simulink model "rp_spectrometer_v2"  (R2022a)
settings: Solver=FixedStepDiscrete  StartTime=0.0  StopTime=4194304  RelTol=1e-3
undefined symbols (not defined in the file): xc7z010clg400
libraries: hdlBasic x93, casper_library_misc x4, vmcUtilities x1, xps_library x1
(part 2 of 2)

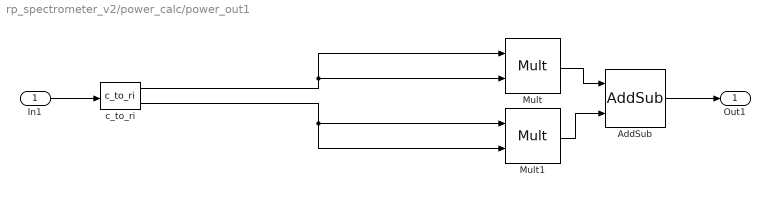
== system rp_spectrometer_v2/power_calc/power_out1 ==
  In1 : Inport
  AddSub : hdlBasic/AddSub  mode=Addition  use_carryin=off  use_carryout=off  en=off  latency=0  precision=Full  arith_type=Unsigned  n_bits=16  bin_pt=14  quantization=Truncate  overflow=Wrap  use_behavioral_HDL=off  hw_selection=Fabric  pipelined=off  XmcBlockStatus=1  maskContainerNames=tabcontainer1  block_type=addsub  block_config=sysgen:Addsub_config
  Mult : hdlBasic/Mult  precision=User Defined  arith_type="Signed  (2's comp)"  n_bits=32  bin_pt=30  quantization=Truncate  overflow=Wrap  en=off  latency=0  use_behavioral_HDL=off  opt=Speed  use_embedded=on  optimum_pipeline=off  pipeline=on  use_rpm=on  placement_style=Triangular  XmcBlockStatus=1  maskContainerNames=group1  block_type=mult  block_config=sysgen:Mult_config  block_width=598  block_height=876
  Mult1 : hdlBasic/Mult  precision=User Defined  arith_type="Signed  (2's comp)"  n_bits=32  bin_pt=30  quantization=Truncate  overflow=Wrap  en=off  latency=0  use_behavioral_HDL=off  opt=Speed  use_embedded=on  optimum_pipeline=off  pipeline=on  use_rpm=on  placement_style=Triangular  XmcBlockStatus=1  maskContainerNames=group1  block_type=mult  block_config=sysgen:Mult_config  block_width=598  block_height=876
  c_to_ri : casper_library_misc/c_to_ri  n_bits=14  bin_pt=13
      settings: AttributesFormatString=14_13 r/i  SourceProductName=CASPER DSP Blockset
  Out1 : Outport  VectorParamsAs1DForOutWhenUnconnected=off
  wires:
  Mult1/1 -> AddSub/2
  Mult/1 -> AddSub/1
  AddSub/1 -> Out1/1
  In1/1 -> c_to_ri/1
  c_to_ri/1 -> Mult/2, Mult/1
  c_to_ri/2 -> Mult1/1, Mult1/2

== system rp_spectrometer_v2/simple_bram_vacc/delay_bram ==
  In1 : Inport
  Constant2 : hdlBasic/Constant  const=1  gui_display_data_type=Boolean  arith_type=Boolean  n_bits=1  bin_pt=0  preci_type=Single  exp_width=8  frac_width=24  explicit_period=on  period=1  XmcBlockStatus=1  maskContainerNames=tabcontainer1  block_type=constant  block_config=sysgen:Constant_config
  Counter : hdlBasic/Counter  cnt_type=Count limited  cnt_to=DelayLen - bram_latency - 1  operation=Up  start_count=0  cnt_by_val=1  arith_type=Unsigned  n_bits=BitWidth  bin_pt=0  load_pin=off  rst=off  en=off  explicit_period=Explicit  period=1  use_behavioral_HDL=off  implementation=Fabric  use_rpm=off  XmcBlockStatus=1  maskContainerNames=group1  block_type=counter  block_config=sysgen:Counter_config  block_width=531  block_height=1023
  Single Port RAM : hdlBasic/Single Port RAM  depth=2^BitWidth  initVector=0  distributed_mem=Block RAM  write_mode=Read Before Write  rst=off  init_reg=0  en=off  optimize_latency=off  latency=bram_latency  optimize=Area  dbl_ovrd=off  simulation_type=fast_sim  XmcBlockStatus=1  maskContainerNames=tabcontainer1  block_type=spram  block_config=sysgen:SPRAM_config
      settings: xl_area=[0, 0, 0, 0, 0, 0, 0]
  Out1 : Outport  VectorParamsAs1DForOutWhenUnconnected=off
  wires:
  Constant2/1 -> Single Port RAM/3
  In1/1 -> Single Port RAM/2
  Counter/1 -> Single Port RAM/1
  Single Port RAM/1 -> Out1/1

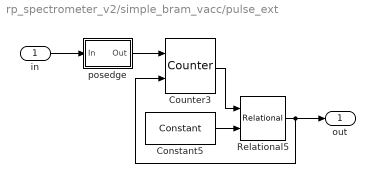
== system rp_spectrometer_v2/simple_bram_vacc/pulse_ext ==
  in : Inport
  Constant5 : hdlBasic/Constant  const=pulse_len  gui_display_data_type=Fixed-point  arith_type=Unsigned  n_bits=bits  bin_pt=0  preci_type=Single  exp_width=8  frac_width=24  explicit_period=off  period=1  XmcBlockStatus=1  maskContainerNames=tabcontainer1  block_type=constant  block_config=sysgen:Constant_config
  Counter3 : hdlBasic/Counter  cnt_type=Free running  cnt_to=1023  operation=Up  start_count=0  cnt_by_val=1  arith_type=Unsigned  n_bits=bits  bin_pt=0  load_pin=off  rst=on  en=on  explicit_period=Explicit  period=1  use_behavioral_HDL=off  implementation=Fabric  use_rpm=on  XmcBlockStatus=1  maskContainerNames=group1  block_type=counter  block_config=sysgen:Counter_config  block_width=531  block_height=1023
  Relational5 : hdlBasic/Relational  mode=a!=b  op_type=Bool  en=off  latency=0  XmcBlockStatus=1  maskContainerNames=tabcontainer1  block_type=relational  block_config=sysgen:Relational_config
  posedge : Subsystem  Tag=Rising Edge Detector
  out : Outport  VectorParamsAs1DForOutWhenUnconnected=off
  wires:
  Counter3/1 -> Relational5/1
  Constant5/1 -> Relational5/2
  Relational5/1 -> Counter3/2, out/1
  in/1 -> posedge/1(In)
  posedge/1(Out) -> Counter3/1

== system rp_spectrometer_v2/simple_bram_vacc1/delay_bram ==
  In1 : Inport
  Constant2 : hdlBasic/Constant  const=1  gui_display_data_type=Boolean  arith_type=Boolean  n_bits=1  bin_pt=0  preci_type=Single  exp_width=8  frac_width=24  explicit_period=on  period=1  XmcBlockStatus=1  maskContainerNames=tabcontainer1  block_type=constant  block_config=sysgen:Constant_config
  Counter : hdlBasic/Counter  cnt_type=Count limited  cnt_to=DelayLen - bram_latency - 1  operation=Up  start_count=0  cnt_by_val=1  arith_type=Unsigned  n_bits=BitWidth  bin_pt=0  load_pin=off  rst=off  en=off  explicit_period=Explicit  period=1  use_behavioral_HDL=off  implementation=Fabric  use_rpm=off  XmcBlockStatus=1  maskContainerNames=group1  block_type=counter  block_config=sysgen:Counter_config  block_width=531  block_height=1023
  Single Port RAM : hdlBasic/Single Port RAM  depth=2^BitWidth  initVector=0  distributed_mem=Block RAM  write_mode=Read Before Write  rst=off  init_reg=0  en=off  optimize_latency=off  latency=bram_latency  optimize=Area  dbl_ovrd=off  simulation_type=fast_sim  XmcBlockStatus=1  maskContainerNames=tabcontainer1  block_type=spram  block_config=sysgen:SPRAM_config
      settings: xl_area=[0, 0, 0, 0, 0, 0, 0]
  Out1 : Outport  VectorParamsAs1DForOutWhenUnconnected=off
  wires:
  Constant2/1 -> Single Port RAM/3
  In1/1 -> Single Port RAM/2
  Counter/1 -> Single Port RAM/1
  Single Port RAM/1 -> Out1/1

== system rp_spectrometer_v2/simple_bram_vacc1/pulse_ext ==
  in : Inport
  Constant5 : hdlBasic/Constant  const=pulse_len  gui_display_data_type=Fixed-point  arith_type=Unsigned  n_bits=bits  bin_pt=0  preci_type=Single  exp_width=8  frac_width=24  explicit_period=off  period=1  XmcBlockStatus=1  maskContainerNames=tabcontainer1  block_type=constant  block_config=sysgen:Constant_config
  Counter3 : hdlBasic/Counter  cnt_type=Free running  cnt_to=1023  operation=Up  start_count=0  cnt_by_val=1  arith_type=Unsigned  n_bits=bits  bin_pt=0  load_pin=off  rst=on  en=on  explicit_period=Explicit  period=1  use_behavioral_HDL=off  implementation=Fabric  use_rpm=on  XmcBlockStatus=1  maskContainerNames=group1  block_type=counter  block_config=sysgen:Counter_config  block_width=531  block_height=1023
  Relational5 : hdlBasic/Relational  mode=a!=b  op_type=Bool  en=off  latency=0  XmcBlockStatus=1  maskContainerNames=tabcontainer1  block_type=relational  block_config=sysgen:Relational_config
  posedge : Subsystem  Tag=Rising Edge Detector
  out : Outport  VectorParamsAs1DForOutWhenUnconnected=off
  wires:
  Counter3/1 -> Relational5/1
  Constant5/1 -> Relational5/2
  Relational5/1 -> Counter3/2, out/1
  in/1 -> posedge/1(In)
  posedge/1(Out) -> Counter3/1

== system rp_spectrometer_v2/simple_bram_vacc/pulse_ext/posedge ==
  In : Inport
  Delay : hdlBasic/Delay  rst=off  en=off  latency=1  reg_retiming=off  XmcBlockStatus=1  maskContainerNames=group1  block_type=delay  block_config=sysgen:Delay_config
  Inverter : hdlBasic/Inverter  en=off  latency=0  XmcBlockStatus=1  maskContainerNames=group2  block_type=inv  block_config=sysgen:Inverter_config
  Logical : hdlBasic/Logical  logical_function=AND  inputs=2  en=off  latency=0  precision=Full  arith_type=Unsigned  n_bits=8  bin_pt=2  align_bp=on  overflow=[]  quantization=[]  XmcBlockStatus=1  maskContainerNames=tabcontainer1  block_type=logical  block_config=sysgen:Logical_config
  Out : Outport  VectorParamsAs1DForOutWhenUnconnected=off
  wires:
  Delay/1 -> Inverter/1
  Inverter/1 -> Logical/1
  In/1 -> Delay/1, Logical/2
  Logical/1 -> Out/1

== system rp_spectrometer_v2/simple_bram_vacc1/pulse_ext/posedge ==
  In : Inport
  Delay : hdlBasic/Delay  rst=off  en=off  latency=1  reg_retiming=off  XmcBlockStatus=1  maskContainerNames=group1  block_type=delay  block_config=sysgen:Delay_config
  Inverter : hdlBasic/Inverter  en=off  latency=0  XmcBlockStatus=1  maskContainerNames=group2  block_type=inv  block_config=sysgen:Inverter_config
  Logical : hdlBasic/Logical  logical_function=AND  inputs=2  en=off  latency=0  precision=Full  arith_type=Unsigned  n_bits=8  bin_pt=2  align_bp=on  overflow=[]  quantization=[]  XmcBlockStatus=1  maskContainerNames=tabcontainer1  block_type=logical  block_config=sysgen:Logical_config
  Out : Outport  VectorParamsAs1DForOutWhenUnconnected=off
  wires:
  Delay/1 -> Inverter/1
  Inverter/1 -> Logical/1
  In/1 -> Delay/1, Logical/2
  Logical/1 -> Out/1
